simulink model "ultrasonic_localization"  (R2024b)
settings: Solver=FixedStepDiscrete  StartTime=0.0  StopTime=60  FixedStep=0.01  RelTol=1e-3
InitFcn:
  | assert(exist('ultraCfg','var')==1,'Run launchUltra first.');
settings Model: Creator=장동민  LastModifiedBy=장동민

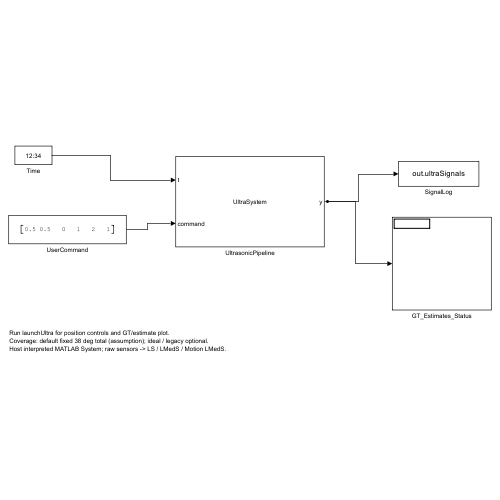
[thumbnail: Simulink's stored preview of the top-level diagram]
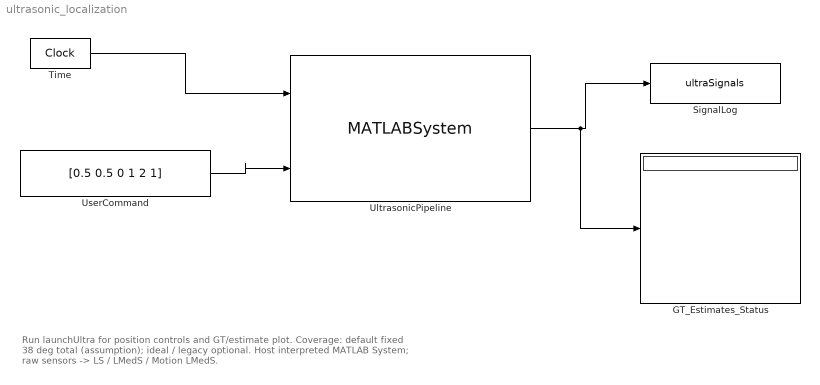
== system ultrasonic_localization ==
  note: Run launchUltra for position controls and GT/estimate plot.
      | Coverage: default fixed 38 deg total (assumption); ideal / legacy optional.
      | Host interpreted MATLAB System; raw sensors -> LS / LMedS / Motion LMedS.
  GT_Estimates_Status : Display
  SignalLog : ToWorkspace  VariableName=ultraSignals  SaveFormat=Timeseries  SampleTime=-1
  Time : DigitalClock  SampleTime=0.01
  UltrasonicPipeline : MATLABSystem  System=UltraSystem  Config=ultraCfg  SimulateUsing=Interpreted execution
      mask Type: UltraSystem
      mask Display:
      | disp('UltraSystem');
      | port_label('input',1,'t');
      | port_label('input',2,'command');
      | port_label('output',1,'y');
  UserCommand : Constant  Value=[0.5 0.5 0 1 2 1]  SampleTime=0.01
  wires:
  Time/1 -> UltrasonicPipeline/1
  UserCommand/1 -> UltrasonicPipeline/2
  UltrasonicPipeline/1 -> SignalLog/1, GT_Estimates_Status/1
